simulink model "elektronikk_model"  (R2025b)
settings: Solver=VariableStepAuto  StartTime=0.0  StopTime=0.1  RelTol=1e-3
libraries: slpidlib x1
settings Model: Creator=vikin  LastModifiedBy=vikin

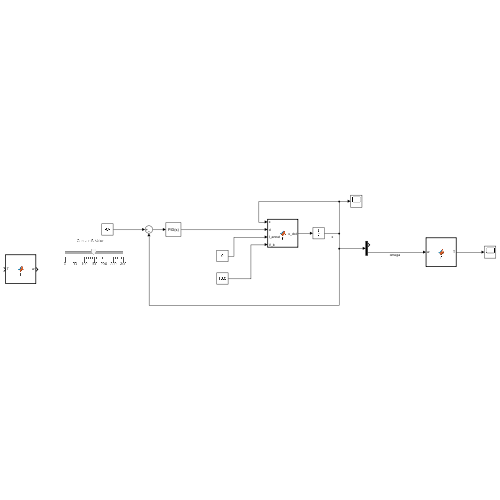
[thumbnail: Simulink's stored preview of the top-level diagram]
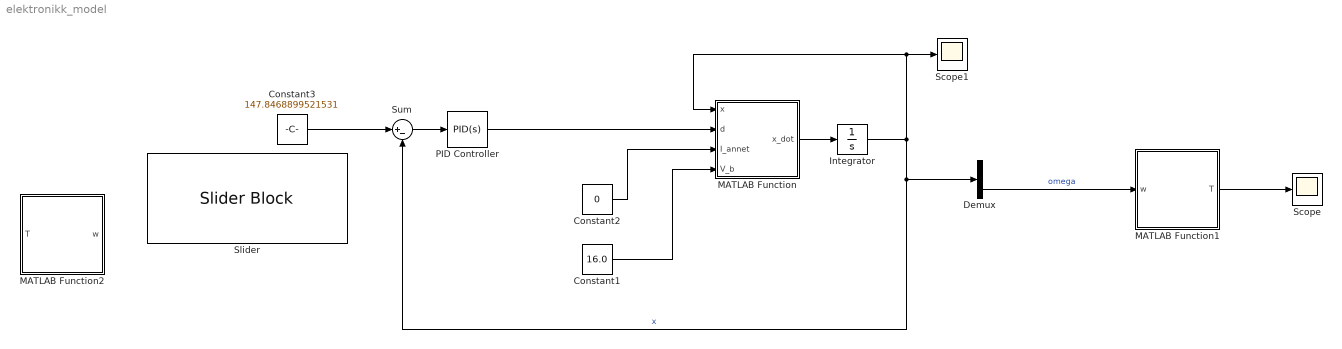
== system elektronikk_model ==
  Constant1 : Constant  Value=16.0
  Constant2 : Constant  Value=0
  Constant3 : Constant  Value=147.8468899521531
  Demux : Demux  Outputs=2
  Integrator : Integrator  InitialCondition=zeros(8,1)
  MATLAB Function : MATLAB Function  TreatAsAtomicUnit=on
  MATLAB Function1 : MATLAB Function  TreatAsAtomicUnit=on
  MATLAB Function2 : MATLAB Function  TreatAsAtomicUnit=on
  PID Controller : slpidlib/PID Controller  Controller=PID  Form=Parallel  TimeDomain=Continuous-time  UseExternalTs=off  SampleTime=-1  IntegratorMethod=Forward Euler  FilterMethod=Forward Euler  ControllerParametersSource=internal  P=1  I=1  UseKiTs=off  D=0  UseExternalDerivativeSource=off  N=100  UseFilter=on  TunerSelectOption=Transfer Function Based (PID Tuner App)  InitialConditionSource=internal  InitialConditionForIntegrator=0  InitialConditionForFilter=0  DifferentiatorICPrevScaledInput=0  ExternalReset=none  TrackingMode=off  Kt=1  LimitOutput=off  SatLimitsSource=internal  UpperSaturationLimit=inf  LowerSaturationLimit=-inf  LinearizeAsGain=on  AntiWindupMode=none  Kb=1  LimitIntegrator=off  UpperIntegratorSaturationLimit=inf  LowerIntegratorSaturationLimit=-inf  POutMin=[]  POutMax=[]  IOutMin=[]  IOutMax=[]  DOutMin=[]  DOutMax=[]  NOutMin=[]  NOutMax=[]  SumOutMin=[]  SumOutMax=[]  SaturationOutMin=[]  SaturationOutMax=[]  PParamMin=[]  PParamMax=[]  IParamMin=[]  IParamMax=[]  DParamMin=[]  DParamMax=[]  NParamMin=[]  NParamMax=[]  KbParamMin=[]  KbParamMax=[]  KtParamMin=[]  KtParamMax=[]  KbOutMin=[]  KbOutMax=[]  KtOutMin=[]  KtOutMax=[]  IntegratorOutMin=[]  IntegratorOutMax=[]  FilterOutMin=[]  FilterOutMax=[]  SumI1OutMin=[]  SumI1OutMax=[]  SumI2OutMin=[]  SumI2OutMax=[]  SumI3OutMin=[]  SumI3OutMax=[]  SumI4OutMin=[]  SumI4OutMax=[]  SumDOutMin=[]  SumDOutMax=[]  DifferentiatorOutMin=[]  DifferentiatorOutMax=[]  FilterDiffOutCoefMin=[]  FilterDiffOutCoefMax=[]  ReciprocalOutMin=[]  ReciprocalOutMax=[]  SumDenOutMin=[]  SumDenOutMax=[]  SumNumOutMin=[]  SumNumOutMax=[]  DivideOutMin=[]  DivideOutMax=[]  UdiffTsProdOutMin=[]  UdiffTsProdOutMax=[]  NTsProdOutMin=[]  NTsProdOutMax=[]  UintegralTsProdOutMin=[]  UintegralTsProdOutMax=[]  UngainTsProdOutMin=[]  UngainTsProdOutMax=[]  ClampingZeroOutDataTypeStr=Inherit: Inherit via back propagation  ClampingZeroOutMin=[]  ClampingZeroOutMax=[]  FilterDenConstantOutDataTypeStr=Inherit: Inherit via back propagation  FilterDenConstantOutMin=[]  FilterDenConstantOutMax=[]  PCopyOutDataTypeStr=Inherit: Inherit via back propagation  PCopyOutMin=[]  PCopyOutMax=[]  NCopyOutDataTypeStr=Inherit: Inherit via back propagation  NCopyOutMin=[]  NCopyOutMax=[]  IntegratorContinuousStateAttributes=''  IntegratorStateMustResolveToSignalObject=off  IntegratorRTWStateStorageClass=Auto  FilterContinuousStateAttributes=''  FilterStateMustResolveToSignalObject=off  FilterRTWStateStorageClass=Auto  ParallelPVariant=InternalParameters  IdealPVariant=Disabled  IVariant=InternalParameters  DVariant=InternalParameters  IntegratorVariant=Continuous  SatVariant=Disabled  AWVariant=Passthrough  PCopyVariant=Disabled  TRVariant=Disabled  FdbkBlocksVariant=Forward  IdealPFdbkVariant=Disabled  SatFdbkVariant=Disabled  DerivativeFilterVariant=ContFilter  NVariant=InternalParameters  NCopyVariant=Disabled  FilterICVariant=InternalICsFilter  IntegratorICVariant=InternalICs  ExternalResetVariant=Disabled  TRSumVariant=Passthrough  SumFdbkVariant=Disabled  SumVariant=Sum_PID  TsampFilterVariant=InternalTs  TsampNgainVariant=Passthrough  TsampIntegralVariant=Disabled_SignalSpec  ExternalSaturationOutDataTypeStr=Inherit: Same as second input  DerivativeSourceVariant=ErrorSignal  PreIntVariant=InternalPreInt
  Scope : Scope
      settings: ActiveDisplayYMinimum=-6.6989381183902221  ActiveDisplayYMaximum=60.290443065512015
  Scope1 : Scope
      settings: ActiveDisplayYMinimum=-416.08103054919775  ActiveDisplayYMaximum=460.14405164058758
  Slider : SliderBlock  ScaleMax=300
  Sum : Sum  Inputs=|+-
  wires:
  MATLAB Function/1(x_dot) -> Integrator/1
  Integrator/1 -> Demux/1, Sum/2, MATLAB Function/1(x), Scope1/1  "x"
  Constant1/1 -> MATLAB Function/4(V_b)
  Constant2/1 -> MATLAB Function/3(I_annet)
  Demux/2 -> MATLAB Function1/1(w)  "omega"
  MATLAB Function1/1(T) -> Scope/1
  Sum/1 -> PID Controller/1
  Constant3/1 -> Sum/1
  PID Controller/1 -> MATLAB Function/2(d)

== matlab function elektronikk_model/MATLAB Function1 ==
  data: w input; T output
function T = f(w)

% Batteri konstanter
R_b = 30*10^-3;

% Ledningskonstanter
R_l = 20*10^-3;
C_l = 100*10^-6;

% DC motor model konstanter
K = 0.020;
R_m = 360*10^-3;
L_m = 154*10^-6;
I_0 = 10*10^-3;
N = 7;

% Propell model konstanter
J_m = 5.85*10^-6;
D = 76*10^-3;
rho = 998; 
% Statisk, J = 0
k_T = 3*10^-4;
k_Q = 3.6 * 10^-6;


T = k_T * w.^2;

== matlab function elektronikk_model/MATLAB Function ==
  data: x input; x_dot output; d input; I_annet input; V_b input
function x_dot = f(x,d,I_annet, V_b)
d = double(d);
x = double(x);

% Batteri konstanter
R_b = 0;%double(30*10^-3);

% Ledningskonstanter
R_l = 0;%20*10^-3;
C_l = 100*10^-6;

% DC motor model konstanter
K = 0.020;
R_m = 360*10^-3;
L_m = double(154*10^-6);
I_0 = 10*10^-3;
N = 7;

% Propell model konstanter
J_m = double(5.85*10^-6);
D = 76*10^-3;
rho = 998; 
% Statisk, J = 0
k_T = 4*10^-4;
k_Q = 3.6 * 10^-6;

x = x(:);            % sikrer 8x1
d = d(:);            % sikrer 4x1

i     = x(1:4);
omega = x(5:8);

a_11 = -(R_m*eye(4) + (R_b + R_l)*(d*d'))/L_m;
a_12 = -K/L_m*eye(4);
a_21 =  K/J_m*eye(4);
a_22 = zeros(4);
A = [a_11 a_12; a_21 a_22];

dw = 0.1;                                  % rad/s, sticking window
i_f = I_0*sign(omega);                     % sliding friction
stuck = abs(omega) < dw;
i_f(stuck) = max(-I_0, min(I_0, i(stuck)));   % cancel i, up to +/-I_0

b_1 = (V_b - R_b*I_annet)/L_m .*d;
b_2 = -(k_Q*omega.*abs(omega) + K*i_f.*sign(omega))/J_m;
B = [b_1; b_2];

x_dot = A*x + B;

== matlab function elektronikk_model/MATLAB Function2 ==
  data: T input; w output
function w = f(T)

% Batteri konstanter
R_b = 30*10^-3;

% Ledningskonstanter
R_l = 20*10^-3;
C_l = 100*10^-6;

% DC motor model konstanter
K = 0.020;
R_m = 360*10^-3;
L_m = 154*10^-6;
I_0 = 10*10^-3;
N = 7;

% Propell model konstanter
J_m = 5.85*10^-6;
D = 76*10^-3;
rho = 998; 
% Statisk, J = 0
k_T = 3*10^-4;
k_Q = 3.6 * 10^-6;


 w =  T/k_T;
